simulink model "fcn2"  (Simulink 7.1)
settings: Solver=VariableStepDiscrete  StartTime=0.0  StopTime=10.0  RelTol=1e-3
settings Model: Creator=W7  LastModifiedBy=W7
settings DataIOCC: ExternalInput=[u]  LoadExternalInput=on
settings DebuggingCC: SolverPrmCheckMsg=none

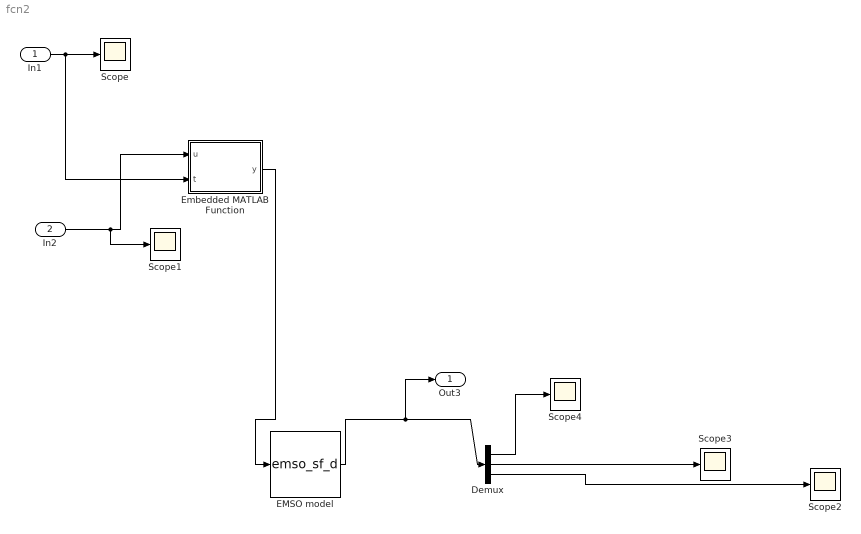
== system fcn2 ==
  In1 : Inport  OutDataType=sfix(16)  OutScaling=2^0
  In2 : Inport  Port=2  OutDataType=sfix(16)  OutScaling=2^0  Interpolate=off
  Demux : Demux  Outputs=3
  EMSO model : S-Function  FunctionName=emso_sf_d  Parameters='Problem_2F2.ems',1,3,0.5  EnableBusSupport=off
  Embedded MATLAB Function : Stateflow chart
  Scope{,1..4} (5 alike) : Scope
      Scope2 settings: TimeRange=5  YMin=0  YMax=45  SaveName=ScopeData4
      Scope3 settings: TimeRange=5  YMin=0  YMax=45  SaveName=ScopeData2
      Scope4 settings: TimeRange=5  YMin=0  YMax=45  SaveName=ScopeData3
  Out3 : Outport
  wires:
  In2/1 -> Embedded MATLAB Function/1(u), Scope1/1
  In1/1 -> Scope/1, Embedded MATLAB Function/2(t)
  EMSO model/1 -> Demux/1, Out3/1
  Demux/3 -> Scope2/1
  Demux/2 -> Scope3/1
  Demux/1 -> Scope4/1
  Embedded MATLAB Function/1(y) -> EMSO model/1

== matlab function Embedded MATLAB Function ==
  data: u input double; y output double; t input double
function y = fcn(u,t)
% This block supports the Embedded MATLAB subset.
% See the help menu for details. 

    y= u;
end
